simulink model "DCDC_Isolated_Step_Up_Converter"  (R2024b)
settings: Solver=VariableStepAuto  StartTime=0.0  StopTime=10.0  RelTol=1e-3
libraries: spsMosfetLib x4, spsVoltageMeasurementLib x3, spsSeriesRLCBranchLib x2, spsCurrentMeasurementLib x2, spsDiodeLib x2, spsDCVoltageSourceLib x1, spsGroundLib x1, spsLinearTransformerLib x1, sps_lib x1
settings Model: Creator=SUDHAK1  LastModifiedBy=SUDHAK1

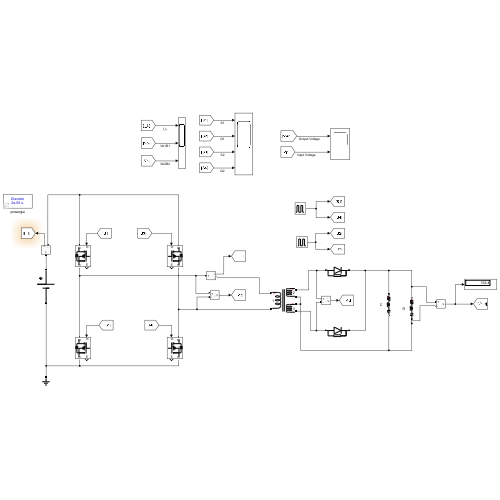
[thumbnail: Simulink's stored preview of the top-level diagram]
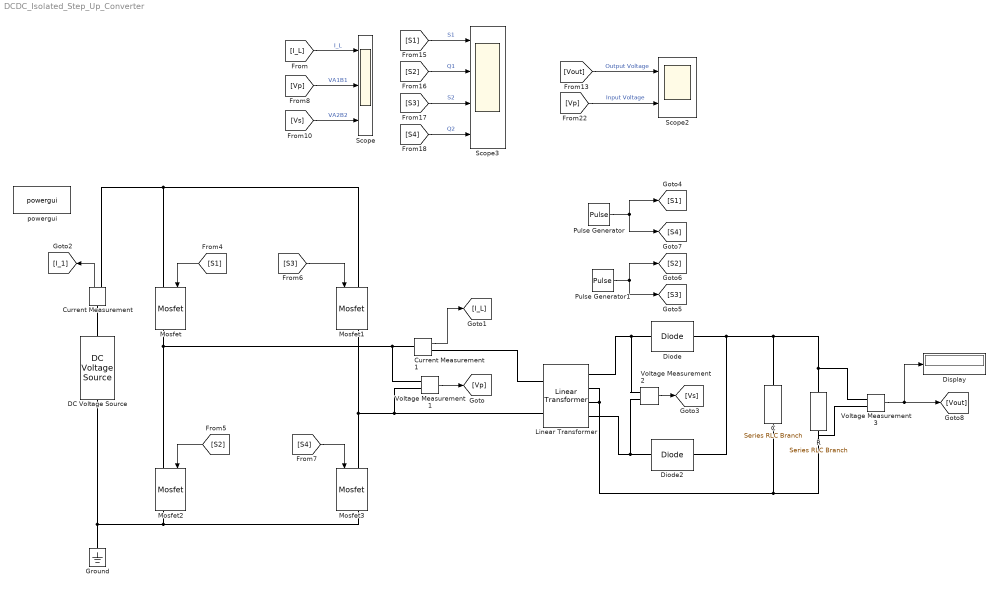
== system DCDC_Isolated_Step_Up_Converter ==
  C : spsSeriesRLCBranchLib/Series RLC Branch  LConnTagsString=__new0  RConnTagsString=__new0  BranchType=RLC  Resistance=1  Inductance=1e-3  SetiL0=off  InitialCurrent=0  Capacitance=100e-6  Setx0=off  InitialVoltage=0  Measurements=None
  Current Measurement : spsCurrentMeasurementLib/Current Measurement  PhasorSimulation=off  OutputType=Complex  PSBequivalent=0
  Current Measurement1 : spsCurrentMeasurementLib/Current Measurement  PhasorSimulation=off  OutputType=Complex  PSBequivalent=0
  DC Voltage Source : spsDCVoltageSourceLib/DC Voltage Source  Amplitude=100  Measurements=None
  Diode : spsDiodeLib/Diode  Ron=0.001  Lon=0  Vf=0.8  IC=0  UseSnubber=0  Rs=500  Cs=250e-9  Measurements=off
  Diode2 : spsDiodeLib/Diode  Ron=0.001  Lon=0  Vf=0.8  IC=0  UseSnubber=0  Rs=500  Cs=250e-9  Measurements=off
  Display : Display
  Ground : spsGroundLib/Ground  LConnTagsString=a
  Linear Transformer : spsLinearTransformerLib/Linear Transformer  UNITS=SI  NominalPower=[50 50]  winding1=[100 0 0]  winding2=[100 0 0]  ThreeWindings=on  winding3=[100 0 0]  RmLm=[9.0038e+09 14330]  Measurements=None  DataType=on
  Mosfet{,1..3} (4 alike) : spsMosfetLib/Mosfet  Ron=0.1  Lon=0  Rd=0.01  Vfd=0  IC=0  Rs=1e5  Cs=inf  Measurements=on
  Pulse Generator : DiscretePulseGenerator  PulseType=Time based  Period=10  PulseWidth=0.02
  Pulse Generator1 : DiscretePulseGenerator  PulseType=Time based  Period=10  PulseWidth=0.02  PhaseDelay=180*0.02/360
  R : spsSeriesRLCBranchLib/Series RLC Branch  LConnTagsString=__new0  RConnTagsString=__new0  BranchType=RLC  Resistance=10  Inductance=1e-3  SetiL0=off  InitialCurrent=0  Capacitance=1e-6  Setx0=off  InitialVoltage=0  Measurements=None
  Scope : Scope  NumInputPorts=3
  Scope2 : Scope  NumInputPorts=2
  Scope3 : Scope  NumInputPorts=4
  Voltage Measurement1 : spsVoltageMeasurementLib/Voltage Measurement  PhasorSimulation=off  OutputType=Complex  PSBequivalent=0
  Voltage Measurement2 : spsVoltageMeasurementLib/Voltage Measurement  PhasorSimulation=off  OutputType=Complex  PSBequivalent=0
  Voltage Measurement3 : spsVoltageMeasurementLib/Voltage Measurement  PhasorSimulation=off  OutputType=Complex  PSBequivalent=0
  powergui : sps_lib/powergui  Priority=1  SimulationMode=Discrete  SampleTime=1/50000  frequency=60  Iterations=50  frequencyindice=0  Pbase=100e6  ErrMax=1e-4  UnitsV=kV  UnitsW=MW  buscounter=0  FunctionMessages=off  echomessages=off  EnableUseOfTLC=off  CurrentSourceSwitches=off  DisableSnubberDevices=off  DisableRonSwitches=off  DisableVfSwitches=off  DisplayEquations=off  AutomaticDiscreteSolvers=off  SolverType=Tustin/Backward Euler (TBE)  Interpol=off  ExternalGateDelay=off  methode=off  Ts=100  x0status=blocks  SPID=on  SwTol=0  HookPort=off  NonlinearTolerance=1e-4  nMaxIteration=100  ContinueOnMaxIteration=off  RestoreLinks=warning  ResistiveCurrentMeasurement=off  Frange=[0:2:500]  Ylog=off  Xlog=on  ShowGrid=off  save=off  variable=ZData  structure=0  ZoomFFT=off  StartTime=0.0  cycles=1  DisplayStyle=1  fundamental=60  FreqAxis=off  MaxFrequency=1000  frequencyindicesteady=1  RmsSteady=1  display=off
  wires:
  [S1] -> Scope3/1  "S1"
  [Vs] -> Scope/3  "VA2B2"
  [S2] -> Mosfet2/1
  [S3] -> Mosfet1/1
  [S4] -> Mosfet3/1
  Voltage Measurement1/1 -> [Vp]
  [S1] -> Mosfet/1
  [S2] -> Scope3/2  "Q1"
  [S4] -> Scope3/4  "Q2"
  [S3] -> Scope3/3  "S2"
  Voltage Measurement2/1 -> [Vs]
  [Vp] -> Scope/2  "VA1B1"
  [I_L] -> Scope/1  "I_L"
  [Vout] -> Scope2/1  "Output Voltage"
  [Vp] -> Scope2/2  "Input Voltage"
  Current Measurement1/1 -> [I_L]
  Current Measurement/1 -> [I_1]
  Pulse Generator/1 -> [S1], [S4]
  Pulse Generator1/1 -> [S3], [S2]
  Voltage Measurement3/1 -> Display/1, [Vout]
  connections:
  Mosfet3/RConn1 -- Mosfet2/RConn1 -- Ground/LConn1 -- DC Voltage Source/LConn1
  Mosfet1/LConn1 -- Mosfet/LConn1 -- Current Measurement/RConn1
  Current Measurement1/LConn1 -- Mosfet/RConn1 -- Mosfet2/LConn1 -- Voltage Measurement1/LConn1
  Mosfet3/LConn1 -- Mosfet1/RConn1 -- Voltage Measurement1/LConn2 -- Linear Transformer/LConn2
  DC Voltage Source/RConn1 -- Current Measurement/LConn1
  Current Measurement1/RConn1 -- Linear Transformer/LConn1
  Linear Transformer/RConn2 -- Voltage Measurement3/LConn2 -- R/RConn1 -- C/RConn1 -- Linear Transformer/RConn3
  Linear Transformer/RConn1 -- Voltage Measurement2/LConn1 -- Diode/LConn1
  Linear Transformer/RConn4 -- Voltage Measurement2/LConn2 -- Diode2/LConn1
  Diode2/RConn1 -- Voltage Measurement3/LConn1 -- R/LConn1 -- C/LConn1 -- Diode/RConn1
